simulink model "system_model_NMPC"  (R2025b)
settings: Solver=ode45  StartTime=0.0  StopTime=40000  MaxStep=1.5  RelTol=1e-9
values from neighbouring files (symbols this model uses):
  a_leader = 6786 *10^3    (= 6786000)    [main_setup.m]
  delta_a_ref = 0    [ControllerPerformance.m]    (also in evaluate_orbit_control.m = expandReference(delta_a_ref, n, 'delta_a_ref'); main_setup.m)
  delta_lambda_ref = 20/a_leader    [ControllerPerformance.m]    (also in evaluate_orbit_control.m = expandReference(delta_lambda_ref, n, 'delta_lambda_ref'); main_setup.m = 2.94724432655e-06)
  earth_radi = 6371*10^3    (= 6371000)    [main_setup.m]
  J2 = 1.08263e-3    (= 0.00108263)    [nmpc_orbit_state.m]
  J_2 = 1.08263 * 10^(-3)    (= 0.00108263)    [main_setup.m]
  Kd_follower = 2*zeta_follower*wn_follower *                [Jx_follower ... (first row only)    [ATTITUDE_INITIALS.m]
  Kd_leader = 2*zeta_leader*wn_leader *              [Jx_leader ... (first row only)    [ATTITUDE_INITIALS.m]
  Kp_follower = [Jx_follower ... (first row only)    [ATTITUDE_INITIALS.m]
  Kp_leader = [Jx_leader ... (first row only)    [ATTITUDE_INITIALS.m]
  m_f = 2    [main_setup.m]
  m_l = 2    [main_setup.m]
  Mmax_follower = [3.2e-3 ... (first row only)    [ATTITUDE_INITIALS.m]
  Mmax_leader = [3.2e-3 ... (first row only)    [ATTITUDE_INITIALS.m]
  mu = G*earth_mass    (= 398589196000000)    [main_setup.m]    (also in nmpc_orbit_state.m)
  rho_leader = mean_rho_500km    (= 7.3e-13)    [main_setup.m]
undefined symbols (not defined in the file or in its folder): beta0_sdre, beta_max_sdre, beta_min_sdre, Q_sdre, R_sdre
libraries: mpclib x1
(part 3 of 3)

== matlab function system_model_NMPC/Model/control sdre/sdre controller ==
  data: x input; x_ref input; Delta_beta output; beta_f output; beta_l output; p input; Q input; R input; beta0 input; beta_min input; beta_max input; K output; A_sdc output; B_sdc output; P output; Delta_beta_raw output; careRelativeResidual output
function [Delta_beta,beta_f,beta_l,K,A_sdc,B_sdc,P,Delta_beta_raw,careRelativeResidual] = ...
    sdre_simulink(x,x_ref,p,Q,R,beta0,beta_min,beta_max)
%#codegen
%SDRE_SIMULINK Four-state differential-drag SDRE for Normal simulation.
% Paste this entire file into a Simulink MATLAB Function block.
% Requires MATLAB, Simulink and Control System Toolbox (CARE).
% This is a function with eight inputs, not a workspace setup script.
%
% Fixed-size REAL DOUBLE inputs (disable variable-size in the block):
% x [4 1] = [delta_a;delta_lambda;delta_e_x;delta_e_y].
% delta_a=(a_f-a_l)/a_l; delta_lambda in radians, continuous angle branch.
% x_ref [4 1] = [0;desired_delta_lambda;0;0], constant between setpoint steps.
% p [5 1] = [a_f;e_f;i_f;omega_f;rho_f], metres/radians/kg per cubic metre.
% Q [4 4] symmetric positive semidefinite; R [1 1] strictly positive.
% beta0, beta_min, beta_max [1 1], m^2/kg, common to both spacecraft.
% Project setup angles are in degrees: convert i_f and omega_f to radians.
%
% Output ports IN ORDER:
% 1 Delta_beta [1 1] = beta_f-beta_l (saturated)
% 2 beta_l [1 1], 3 beta_f [1 1], 4 K [1 4], 5 A_sdc [4 4],
% 6 B_sdc [4 1], 7 P [4 4], 8 Delta_beta_raw [1 1],
% 9 careRelativeResidual [1 1]. Terminate unused output ports.
% Connect ports 2 and 3 to U=[beta_l;beta_f]; set U Outport dimension to 2.
%
% Preserves the uploaded sdre.m SDC equations and fixed-mean allocation.
% Assumes zero relative inclination components. Evaluate SDC at x, not error.
% A_sdc(:,2)=0, so A_sdc*x_ref=0 for the supported constant reference.
% Circular/singular eccentricities are excluded, not clipped.
% Invalid inputs or failed CARE stop simulation; no hidden fallback is used.
% CARE runs in MATLAB via an extrinsic call and needs the MATLAB engine.
% Not intended for standalone generated code or deployment.
% Frozen-state CARE checks do not prove saturated trajectory convergence.
%
% If attitude is active, run main_setup BEFORE ATTITUDE_INITIALS because
% main_setup clears the workspace, or comment out the attitude subsystem.
% Disconnecting its input does not exclude it from Simulink compilation.

coder.extrinsic('care');
% A typed, fixed-size destination converts CARE's mxArray output to double.
P = zeros(4,4);
K = zeros(1,4);
Delta_beta = 0.0;
beta_l = 0.0;
beta_f = 0.0;
Delta_beta_raw = 0.0;
careRelativeResidual = 0.0;

%% Input validation.
validateattributes(x,{'double'},{'real','finite','size',[4 1]},mfilename,'x');
validateattributes(x_ref,{'double'},{'real','finite','size',[4 1]},mfilename,'x_ref');
if any(x_ref([1 3 4]) ~= 0)
    error('sdre_fanebust:UnsupportedReference', ...
        'Use x_ref=[0;delta_lambda_desired;0;0] for constant-separation tracking.');
end
tracking_error = x-x_ref;
if any(~isfinite(tracking_error))
    error('sdre_fanebust:NonfiniteError','Tracking error overflow: check x and x_ref.');
end
validateattributes(p,{'double'},{'real','finite','size',[5 1]},mfilename,'p');
validateattributes(Q,{'double'},{'real','finite','size',[4 4]},mfilename,'Q');
validateattributes(R,{'double'},{'real','finite','scalar','positive'},mfilename,'R');
validateattributes(beta0,{'double'},{'real','finite','scalar','nonnegative'});
validateattributes(beta_min,{'double'},{'real','finite','scalar','nonnegative'});
validateattributes(beta_max,{'double'},{'real','finite','scalar','nonnegative'});
if beta_min > beta0 || beta0 > beta_max
    error('sdre_fanebust:Bounds','Require beta_min <= beta0 <= beta_max.');
end
qScale = max(norm(Q,'fro'),realmin);
if norm(Q-Q.','fro') > 1e-12*qScale
    error('sdre_fanebust:QSymmetry','Q must be symmetric.');
end
Q = (Q+Q.')/2;
if min(real(eig(Q))) < -1e-12*qScale
    error('sdre_fanebust:QPositive','Q must be positive semidefinite.');
end

%% Fanebust quantities (A is a scalar, distinct from matrix A_sdc).
a_f = p(1); e_f = p(2); i_f = p(3); omega_f = p(4); rho_f = p(5);
singularityTol = 1e-10;  % Dimensionless exclusion margin, not clipping.
careResidualTol = 1e-8;  % Relative residual threshold.
if a_f <= 0 || e_f <= singularityTol || e_f >= 1-singularityTol ...
        || rho_f < 0 || 1+x(1) <= singularityTol
    error('sdre_fanebust:Domain', ...
        'Require a_f>0, tol<e_f<1-tol, rho_f>=0, and 1+delta_a>tol.');
end
mu = 6.6743e-11*5.972e24;  % Same constants as the original plant.
J2 = 1.08263e-3;
R_E = 6371e3;
A = (3/2)*sqrt(((1+x(1))^7*mu)/a_f^7);
I = 3+5*cos(2*i_f);       % delta_i_x = 0.
Jstar = J2*R_E^2;
c = cos(omega_f); s = sin(omega_f);
% E^2 = e_f^2+x(3)^2+x(4)^2-2*e_f*(x(3)*c+x(4)*s).
% The equivalent hypot form avoids cancellation of expanded terms.
E = hypot(x(3)-e_f*c,x(4)-e_f*s);
if E <= singularityTol || E >= 1-singularityTol || E+e_f <= singularityTol
    error('sdre_fanebust:ESingularity', ...
        'Require tol<E<1-tol and E+e_f>tol; singular denominators are not clipped.');
end
f = 1.61e4*e_f^0.02701-1.61e4; % Original expression and sign.
Gamma = f*rho_f;
G_x = (x(3)-2*e_f*c)/(E+e_f);
G_y = (x(4)-2*e_f*s)/(E+e_f);
% Exact identity: E-e_f = G_x*x(3)+G_y*x(4).

%% Exact four-state SDC matrices, including nominal beta0 in the drift.
h = beta0*(1+x(1))*Gamma/((1-e_f)*(E-1));
d = beta0*Gamma/E;
A_sdc = zeros(4);
A_sdc(1,3) = h*G_x;
A_sdc(1,4) = h*G_y;
A_sdc(2,1) = -A*a_f^2/(1+x(1))^2;
A_sdc(3,3) = d*(1+c*G_x);
A_sdc(3,4) = -(1/4)*Jstar*A*I+d*c*G_y;
A_sdc(4,3) = +(1/4)*Jstar*A*I+d*s*G_x;
A_sdc(4,4) = d*(1+s*G_y);

% Input signs follow directly from beta_l=beta0-Delta_beta/2.
B_sdc = zeros(4,1);
B_sdc(1) = (1/2)*(1+x(1))*Gamma*(1/(1-e_f)-1/(E-1));
B_sdc(3) = (1/2)*Gamma*(c-(x(3)-e_f*c)/E);
B_sdc(4) = (1/2)*Gamma*(s-(x(4)-e_f*s)/E);
if any(~isfinite([A_sdc(:);B_sdc(:);A;I;Jstar;E;f]))
    error('sdre_fanebust:NonfiniteModel','Model overflow: check state/parameter scales.');
end

%% Solve and verify the four-state continuous-time Riccati equation.
% A_sdc'*P + P*A_sdc - P*B_sdc/R*B_sdc'*P + Q = 0.
P = care(A_sdc,B_sdc,Q,R);
if any(~isfinite(P(:)))
    error('sdre_simulink:InvalidCARE','CARE returned a nonfinite solution.');
end
P = (P+P.')/2;
K = (B_sdc.'*P)/R;
poles = eig(A_sdc-B_sdc*K);
t1 = A_sdc.'*P;
t2 = P*A_sdc;
t3 = P*B_sdc*K;
residual = t1+t2-t3+Q;
scale = max(norm(t1,'fro')+norm(t2,'fro')+norm(t3,'fro')+norm(Q,'fro'),realmin);
careRelativeResidual = norm(residual,'fro')/scale;
if ~isfinite(careRelativeResidual) || careRelativeResidual > careResidualTol ...
        || any(~isfinite(poles)) || any(real(poles) >= 0) ...
        || min(real(eig(P))) < -1e-10*max(norm(P,2),realmin)
    error('sdre_simulink:InvalidCARE', ...
        'CARE failed residual, positive-semidefinite, or stable-pole checks.');
end

%% Reference tracking and symmetric physical allocation.
% K comes from the actual-state SDC matrices; feedback acts on x-x_ref.
raw = -(R\(B_sdc.'*P*tracking_error));
if ~isfinite(raw)
    error('sdre_fanebust:InvalidCommand','Nonfinite SDRE command.');
end
% Intersection of both satellites' constraints with fixed mean beta0.
limit = 2*min(beta0-beta_min,beta_max-beta0);
Delta_beta = min(max(raw,-limit),limit);
beta_l = beta0-Delta_beta/2;
beta_f = beta0+Delta_beta/2;

Delta_beta_raw = raw;
end

== matlab function system_model_NMPC/Model/Attitude follower /Attitude Follower/MATLAB Function1 ==
  data: quat input; Euler output; Theta output
function [Euler,Theta] = QToTheta(quat)
quat=quat';
Euler = quat2eul( quat );
Theta = Euler(2);
end

== matlab function system_model_NMPC/Model/Attitude follower /Attitude Follower/PID Follower ==
  data: theta_cmd input; Mb output; attitude_zyx input; pqr input; Kp input; Kd input; Mmax input; angle_error output; Mb_raw output
function [Mb, angle_error, Mb_raw] = attitude_pd_controller( ...
    theta_cmd, attitude_zyx, pqr, Kp, Kd, Mmax)
%ATTITUDE_PD_CONTROLLER Spacecraft attitude PD control with torque limits.
%#codegen
%
% Suitable for a Simulink MATLAB Function block. Configure theta_cmd as
% a scalar and all other inputs as fixed-size [3 1] real double vectors.
% All outputs are fixed-size [3 1] column vectors.
%
% INPUTS
%   theta_cmd    Desired pitch [rad]; desired roll and yaw are zero.
%   attitude_zyx Measured ZYX Euler angles [yaw; pitch; roll] [rad].
%   pqr          Body angular rates [p; q; r] [rad/s].
%   Kp           Proportional gains [roll; pitch; yaw] [N*m/rad].
%   Kd           Derivative gains [roll; pitch; yaw] [N*m*s/rad].
%   Mmax         Nonnegative torque limits [roll; pitch; yaw] [N*m].
%
% OUTPUTS (body-axis order: roll/x, pitch/y, yaw/z)
%   Mb           Saturated commanded body torque [N*m].
%   angle_error  Wrapped measured-minus-command Euler errors [rad].
%   Mb_raw       Unsaturated commanded body torque [N*m].
%
% ASSUMPTIONS
%   Inputs are finite; gains and limits are nonnegative. Body rates are
%   measured relative to the attitude reference frame (e.g. LVLH), and
%   desired relative body rates are zero. No command-rate feedforward is
%   included. Body rates are not generally equal to Euler angle rates.
%   This componentwise Euler PD law is intended for operation away from
%   the ZYX Euler singularity at pitch = +/-pi/2; it is not a global
%   attitude controller. Wrapping each error does not remove that
%   singularity.

% Allocate fixed-size column outputs for MATLAB Coder / Simulink.
Mb = zeros(3, 1);
angle_error = zeros(3, 1);
Mb_raw = zeros(3, 1);

% Reorder [yaw; pitch; roll] into body-axis [roll; pitch; yaw],
% then subtract the command [0; theta_cmd; 0]. Explicit indexing
% avoids implicit expansion and preserves fixed-size column handling.
error_unwrapped = zeros(3, 1);
error_unwrapped(1) = attitude_zyx(3);
error_unwrapped(2) = attitude_zyx(2) - theta_cmd;
error_unwrapped(3) = attitude_zyx(1);

for axis = 1:3
    % Wrap measured-minus-command error to [-pi, pi].
    angle_error(axis) = atan2(sin(error_unwrapped(axis)), ...
                             cos(error_unwrapped(axis)));

    % Componentwise equivalent of -Kp.*angle_error - Kd.*pqr.
    Mb_raw(axis) = -Kp(axis) * angle_error(axis) ...
                  -Kd(axis) * pqr(axis);

    % Independently saturate each body torque to +/-Mmax(axis).
    Mb(axis) = min(max(Mb_raw(axis), -Mmax(axis)), Mmax(axis));
end
end

== matlab function system_model_NMPC/Model/control sdre/P vector ==
  data: x_f input; P output; rho input
function P = parameter_vector(x_f, rho)
% NMPC_PARAMETER_VECTOR
% Creates the parameter vector used by nmpc_orbit_state.
%
% INPUT:
%   x_f(1) = follower semi-major axis, a_f      [m]
%   x_f(2) = follower eccentricity, e_f         [-]
%   x_f(3) = follower inclination, i_f          [rad]
%   x_f(4) = follower argument of periapsis     [rad]
%   x_f(5) = follower RAAN                      [rad]
%   x_f(6) = follower mean anomaly              [rad]
%
%   rho    = atmospheric density                [kg/m^3]
%
% OUTPUT:
%
%   P = [a_f;
%        e_f;
%        i_f;
%        omega_f;
%        rho]

%#codegen

P = zeros(5,1);

P(1) = x_f(1);     % a_f
P(2) = x_f(2);     % e_f
P(3) = x_f(3);     % i_f
P(4) = x_f(4);     % omega_f
P(5) = rho;        % atmospheric density

end

== matlab function system_model_NMPC/Model/control sdre/X vector ==
  data: x input; X output
function X = X_vector(x)
% NMPC_PARAMETER_VECTOR
% Creates the parameter vector used by nmpc_orbit_state.
%
% INPUT:
%   x(1) = delta_a      
%   x(2) = delta_lambda         
%   x(3) = delta_e_x       
%   x(4) = delta_e_y     
%   x(5) = delta_i_x                     [rad]
%   x(6) = delta_i_y                     [rad]
%
% OUTPUT:
%
%   X = [delta_a; delta_lambda; delta_e_x; delta_e_y], size 4-by-1.


X = zeros(4,1);

X(1) = x(1);     
X(2) = x(2);     
X(3) = x(3);     
X(4) = x(4);     

end

== matlab function system_model_NMPC/Model/orbit_Propegation/Beta Follower ==
  data: theta input; beta output; C_d output; A output
function [beta,C_d,A] = theta_to_beta(theta)
% THETA_TO_BETA  Convert a satellite pitch angle theta [rad]
% to the corresponding ballistic coefficient beta [m^2/kg].
%
% 
%
%   This is a direct forward evaluation (no lookup/interpolation needed,
%   since beta(theta) is single-valued) using the same flat-plate /
%   area model as beta_to_theta's table build.

    m = 2; % spacecraft mass [kg]
    
     % Clamp theta
    theta_min = 0;
    theta_max = 83.6557*pi/180;   % [rad], peak of beta(theta)
    theta = min(max(theta, theta_min), theta_max);
    
    % C_d model constant (NRLMSISE-00 based)
    alpha = (7.5*10^(-17)*5.14*10^7*10^6*1011) / (1.0 + (7.5*10^(-17)*5.14*10^7*10^6*1011));
    r = sqrt(1-alpha);

    %theta pitch of satellite [rad]

    % flat plate at incidence theta
    C_d_flat_theta     = 2*(1+(2/3)*r*sin(theta));
    C_d_flat_theta_inv = 2*(1+(2/3)*r*sin(pi/2-theta));

    % Areas
    % 2 solar panels
    A_tot_solar = 2*15*15/10^4;
    A_ref_solar = A_tot_solar*sin(theta);

    % box (front and upper side)
    A_tot_box_front = 10*10/10^4;
    A_tot_box_top   = 15*10/10^4;

    A_ref_box_front = A_tot_box_front*cos(theta);
    A_ref_box_top   = A_tot_box_top*sin(theta);

    A = A_ref_solar + A_ref_box_top + A_ref_box_front;

    % Total drag coefficient (area-weighted blend)
    C_d = (A_ref_box_front/A)*C_d_flat_theta_inv ...
              + ((A-A_ref_box_front)/A)*C_d_flat_theta;

    beta = (A * C_d) / m;

end

== matlab function system_model_NMPC/Model/orbit_Propegation/Beta Leader ==
  data: theta input; beta output; C_d output; A output
function [beta,C_d,A] = theta_to_beta(theta)
% THETA_TO_BETA  Convert a satellite pitch angle theta [rad]
% to the corresponding ballistic coefficient beta [m^2/kg].
%
% 
%
%   This is a direct forward evaluation (no lookup/interpolation needed,
%   since beta(theta) is single-valued) using the same flat-plate /
%   area model as beta_to_theta's table build.

    m = 2; % spacecraft mass [kg]
    
     % Clamp theta
    theta_min = 0;
    theta_max = 83.6557*pi/180;   % [rad], peak of beta(theta)
    theta = min(max(theta, theta_min), theta_max);
    
    % C_d model constant (NRLMSISE-00 based)
    alpha = (7.5*10^(-17)*5.14*10^7*10^6*1011) / (1.0 + (7.5*10^(-17)*5.14*10^7*10^6*1011));
    r = sqrt(1-alpha);
    
    %theta pitch of satellite [rad]

    % flat plate at incidence theta
    C_d_flat_theta     = 2*(1+(2/3)*r*sin(theta));
    C_d_flat_theta_inv = 2*(1+(2/3)*r*sin(pi/2-theta));

    % Areas
    % 2 solar panels
    A_tot_solar = 2*15*15/10^4;
    A_ref_solar = A_tot_solar*sin(theta);

    % box (front and upper side)
    A_tot_box_front = 10*10/10^4;
    A_tot_box_top   = 15*10/10^4;

    A_ref_box_front = A_tot_box_front*cos(theta);
    A_ref_box_top   = A_tot_box_top*sin(theta);

    A = A_ref_solar + A_ref_box_top + A_ref_box_front;

    % Total drag coefficient (area-weighted blend)
    C_d = (A_ref_box_front/A)*C_d_flat_theta_inv ...
              + ((A-A_ref_box_front)/A)*C_d_flat_theta;

    beta = (A * C_d) / m;

end
